simulink model "snap_adc5g_spec"  (R2019a)
settings: Solver=VariableStepDiscrete  StartTime=0.0  StopTime=10.0  RelTol=1e-3
undefined symbols (not defined in the file): pfb_coeff_gen_calc
libraries: xbsIndex_r4 x13965, casper_library_misc x80, casper_library_delays x43, xps_library x5, xbsReplacements_r4 x2, casper_library_communications x1
(part 53 of 152)

== system snap_adc5g_spec/fft_wideband_real/fft_direct/butterfly0_0/bus_convert/conv4 ==
  din : Inport
  all_0s : xbsIndex_r4/Logical  logical_function=NAND  inputs=3  en=off  latency=1  precision=Full  arith_type=Unsigned  n_bits=16  bin_pt=0  align_bp=on  dbl_ovrd=off  block_type=logical
  all_1s : xbsIndex_r4/Logical  logical_function=NAND  inputs=3  en=off  latency=1  precision=Full  arith_type=Unsigned  n_bits=16  bin_pt=0  align_bp=on  dbl_ovrd=off  block_type=logical
  and : xbsIndex_r4/Logical  logical_function=AND  inputs=2  en=off  latency=0  precision=Full  arith_type=Unsigned  n_bits=16  bin_pt=0  align_bp=on  dbl_ovrd=off  block_type=logical
  convert : Subsystem  AncestorBlock=casper_library_misc/convert  mask(convert){bin_pt_in=binary_point_i, n_bits_out=bit_width_o, bin_pt_out=binary_point_o, quantization=Round  (unbiased: Even Values), overflow=Wrap, csp_latency=csp_latency}
      mask prompts: bin_pt_in "Binary Point In"; n_bits_out "Bit Width Out"; bin_pt_out "Binary Point Out"; csp_latency "Latency"
      mask help:
      | Convert input value to the specified bit width and precision.
      |
      | Does not support upscaling number of fractional bits (eg 8_5 to 8_4 is ok, but not 8_4 to 8_5).
      mask init: same as snap_adc5g_spec/fft_wideband_real/fft_direct/butterfly0_0/bus_norm1/conv1
      settings: AttributesFormatString=|
      | N_18 ==> 18_17
      | round even, wrap
      | latency = 1
      mask Help:
      | <pre>
      | Description::
      | 
      | Outputs converted version of the input.
      | 
      | Mask Parameters::
      | 
      | Binary Point In (bin_pt_in): Specifies the binary point location in the input.
      | 
      | Bit Width Out (n_bits_out): Specifies the width of the output.
      | 
      | Binary Point Out (bin_pt_out): Specifies the binary point location in the output.
      | 
      | Quantization (quantization): Specifies quantization handling.
      | 
      | Overflow (overflow): Specifies overflow handling.
      | 
      | Latency (latency): Specifies the latency of the underlying adder block, which is the overall
      | latency of this block as well.
      | </pre>
      mask TypeOptions quantization: Truncate | Round  (unbiased: +/- Inf) | Round  (unbiased: Even Values) | Round  (unbiased: Zero) | Round  (unbiased: Odd Values) | Round  (biased: Up) | Round  (biased: Down)
      mask TypeOptions overflow: Wrap | Saturate | Error
  invert1 : xbsIndex_r4/Inverter  en=off  latency=0  dbl_ovrd=off  block_type=inv
  invert2 : xbsIndex_r4/Inverter  en=off  latency=0  dbl_ovrd=off  block_type=inv
  invert3 : xbsIndex_r4/Inverter  en=off  latency=0  dbl_ovrd=off  block_type=inv
  slice1 : xbsIndex_r4/Slice  nbits=1  boolean_output=on  mode=Upper Bit Location + Width  bit1=0  base1=MSB of Input  bit0=0  base0=LSB of Input  dbl_ovrd=off  block_type=slice
  slice2 : xbsIndex_r4/Slice  nbits=1  boolean_output=on  mode=Upper Bit Location + Width  bit1=-1  base1=MSB of Input  bit0=0  base0=LSB of Input  dbl_ovrd=off  block_type=slice
  slice3 : xbsIndex_r4/Slice  nbits=1  boolean_output=on  mode=Upper Bit Location + Width  bit1=-2  base1=MSB of Input  bit0=0  base0=LSB of Input  dbl_ovrd=off  block_type=slice
  dout : Outport
  of : Outport  Port=2
  wires:
  din/1 -> convert/1(in), slice1/1, slice2/1, slice3/1
  convert/1(out) -> dout/1
  slice1/1 -> all_1s/1, invert1/1
  invert1/1 -> all_0s/1
  slice2/1 -> all_1s/2, invert2/1
  invert2/1 -> all_0s/2
  slice3/1 -> all_1s/3, invert3/1
  invert3/1 -> all_0s/3
  all_0s/1 -> and/1
  all_1s/1 -> and/2
  and/1 -> of/1

== system snap_adc5g_spec/fft_wideband_real/fft_direct/butterfly0_0/bus_convert/conv5 ==
  din : Inport
  all_0s : xbsIndex_r4/Logical  logical_function=NAND  inputs=3  en=off  latency=1  precision=Full  arith_type=Unsigned  n_bits=16  bin_pt=0  align_bp=on  dbl_ovrd=off  block_type=logical
  all_1s : xbsIndex_r4/Logical  logical_function=NAND  inputs=3  en=off  latency=1  precision=Full  arith_type=Unsigned  n_bits=16  bin_pt=0  align_bp=on  dbl_ovrd=off  block_type=logical
  and : xbsIndex_r4/Logical  logical_function=AND  inputs=2  en=off  latency=0  precision=Full  arith_type=Unsigned  n_bits=16  bin_pt=0  align_bp=on  dbl_ovrd=off  block_type=logical
  convert : Subsystem  AncestorBlock=casper_library_misc/convert  mask(convert){bin_pt_in=binary_point_i, n_bits_out=bit_width_o, bin_pt_out=binary_point_o, quantization=Round  (unbiased: Even Values), overflow=Wrap, csp_latency=csp_latency}
      mask prompts: bin_pt_in "Binary Point In"; n_bits_out "Bit Width Out"; bin_pt_out "Binary Point Out"; csp_latency "Latency"
      mask help:
      | Convert input value to the specified bit width and precision.
      |
      | Does not support upscaling number of fractional bits (eg 8_5 to 8_4 is ok, but not 8_4 to 8_5).
      mask init: same as snap_adc5g_spec/fft_wideband_real/fft_direct/butterfly0_0/bus_norm1/conv1
      settings: AttributesFormatString=|
      | N_18 ==> 18_17
      | round even, wrap
      | latency = 1
      mask Help:
      | <pre>
      | Description::
      | 
      | Outputs converted version of the input.
      | 
      | Mask Parameters::
      | 
      | Binary Point In (bin_pt_in): Specifies the binary point location in the input.
      | 
      | Bit Width Out (n_bits_out): Specifies the width of the output.
      | 
      | Binary Point Out (bin_pt_out): Specifies the binary point location in the output.
      | 
      | Quantization (quantization): Specifies quantization handling.
      | 
      | Overflow (overflow): Specifies overflow handling.
      | 
      | Latency (latency): Specifies the latency of the underlying adder block, which is the overall
      | latency of this block as well.
      | </pre>
      mask TypeOptions quantization: Truncate | Round  (unbiased: +/- Inf) | Round  (unbiased: Even Values) | Round  (unbiased: Zero) | Round  (unbiased: Odd Values) | Round  (biased: Up) | Round  (biased: Down)
      mask TypeOptions overflow: Wrap | Saturate | Error
  invert1 : xbsIndex_r4/Inverter  en=off  latency=0  dbl_ovrd=off  block_type=inv
  invert2 : xbsIndex_r4/Inverter  en=off  latency=0  dbl_ovrd=off  block_type=inv
  invert3 : xbsIndex_r4/Inverter  en=off  latency=0  dbl_ovrd=off  block_type=inv
  slice1 : xbsIndex_r4/Slice  nbits=1  boolean_output=on  mode=Upper Bit Location + Width  bit1=0  base1=MSB of Input  bit0=0  base0=LSB of Input  dbl_ovrd=off  block_type=slice
  slice2 : xbsIndex_r4/Slice  nbits=1  boolean_output=on  mode=Upper Bit Location + Width  bit1=-1  base1=MSB of Input  bit0=0  base0=LSB of Input  dbl_ovrd=off  block_type=slice
  slice3 : xbsIndex_r4/Slice  nbits=1  boolean_output=on  mode=Upper Bit Location + Width  bit1=-2  base1=MSB of Input  bit0=0  base0=LSB of Input  dbl_ovrd=off  block_type=slice
  dout : Outport
  of : Outport  Port=2
  wires:
  din/1 -> convert/1(in), slice1/1, slice2/1, slice3/1
  convert/1(out) -> dout/1
  slice1/1 -> all_1s/1, invert1/1
  invert1/1 -> all_0s/1
  slice2/1 -> all_1s/2, invert2/1
  invert2/1 -> all_0s/2
  slice3/1 -> all_1s/3, invert3/1
  invert3/1 -> all_0s/3
  all_0s/1 -> and/1
  all_1s/1 -> and/2
  and/1 -> of/1

== system snap_adc5g_spec/fft_wideband_real/fft_direct/butterfly0_0/bus_convert/conv6 ==
  din : Inport
  all_0s : xbsIndex_r4/Logical  logical_function=NAND  inputs=3  en=off  latency=1  precision=Full  arith_type=Unsigned  n_bits=16  bin_pt=0  align_bp=on  dbl_ovrd=off  block_type=logical
  all_1s : xbsIndex_r4/Logical  logical_function=NAND  inputs=3  en=off  latency=1  precision=Full  arith_type=Unsigned  n_bits=16  bin_pt=0  align_bp=on  dbl_ovrd=off  block_type=logical
  and : xbsIndex_r4/Logical  logical_function=AND  inputs=2  en=off  latency=0  precision=Full  arith_type=Unsigned  n_bits=16  bin_pt=0  align_bp=on  dbl_ovrd=off  block_type=logical
  convert : Subsystem  AncestorBlock=casper_library_misc/convert  mask(convert){bin_pt_in=binary_point_i, n_bits_out=bit_width_o, bin_pt_out=binary_point_o, quantization=Round  (unbiased: Even Values), overflow=Wrap, csp_latency=csp_latency}
      mask prompts: bin_pt_in "Binary Point In"; n_bits_out "Bit Width Out"; bin_pt_out "Binary Point Out"; csp_latency "Latency"
      mask help:
      | Convert input value to the specified bit width and precision.
      |
      | Does not support upscaling number of fractional bits (eg 8_5 to 8_4 is ok, but not 8_4 to 8_5).
      mask init: same as snap_adc5g_spec/fft_wideband_real/fft_direct/butterfly0_0/bus_norm1/conv1
      settings: AttributesFormatString=|
      | N_18 ==> 18_17
      | round even, wrap
      | latency = 1
      mask Help:
      | <pre>
      | Description::
      | 
      | Outputs converted version of the input.
      | 
      | Mask Parameters::
      | 
      | Binary Point In (bin_pt_in): Specifies the binary point location in the input.
      | 
      | Bit Width Out (n_bits_out): Specifies the width of the output.
      | 
      | Binary Point Out (bin_pt_out): Specifies the binary point location in the output.
      | 
      | Quantization (quantization): Specifies quantization handling.
      | 
      | Overflow (overflow): Specifies overflow handling.
      | 
      | Latency (latency): Specifies the latency of the underlying adder block, which is the overall
      | latency of this block as well.
      | </pre>
      mask TypeOptions quantization: Truncate | Round  (unbiased: +/- Inf) | Round  (unbiased: Even Values) | Round  (unbiased: Zero) | Round  (unbiased: Odd Values) | Round  (biased: Up) | Round  (biased: Down)
      mask TypeOptions overflow: Wrap | Saturate | Error
  invert1 : xbsIndex_r4/Inverter  en=off  latency=0  dbl_ovrd=off  block_type=inv
  invert2 : xbsIndex_r4/Inverter  en=off  latency=0  dbl_ovrd=off  block_type=inv
  invert3 : xbsIndex_r4/Inverter  en=off  latency=0  dbl_ovrd=off  block_type=inv
  slice1 : xbsIndex_r4/Slice  nbits=1  boolean_output=on  mode=Upper Bit Location + Width  bit1=0  base1=MSB of Input  bit0=0  base0=LSB of Input  dbl_ovrd=off  block_type=slice
  slice2 : xbsIndex_r4/Slice  nbits=1  boolean_output=on  mode=Upper Bit Location + Width  bit1=-1  base1=MSB of Input  bit0=0  base0=LSB of Input  dbl_ovrd=off  block_type=slice
  slice3 : xbsIndex_r4/Slice  nbits=1  boolean_output=on  mode=Upper Bit Location + Width  bit1=-2  base1=MSB of Input  bit0=0  base0=LSB of Input  dbl_ovrd=off  block_type=slice
  dout : Outport
  of : Outport  Port=2
  wires:
  din/1 -> convert/1(in), slice1/1, slice2/1, slice3/1
  convert/1(out) -> dout/1
  slice1/1 -> all_1s/1, invert1/1
  invert1/1 -> all_0s/1
  slice2/1 -> all_1s/2, invert2/1
  invert2/1 -> all_0s/2
  slice3/1 -> all_1s/3, invert3/1
  invert3/1 -> all_0s/3
  all_0s/1 -> and/1
  all_1s/1 -> and/2
  and/1 -> of/1

== system snap_adc5g_spec/fft_wideband_real/fft_direct/butterfly0_0/bus_convert/conv7 ==
  din : Inport
  all_0s : xbsIndex_r4/Logical  logical_function=NAND  inputs=3  en=off  latency=1  precision=Full  arith_type=Unsigned  n_bits=16  bin_pt=0  align_bp=on  dbl_ovrd=off  block_type=logical
  all_1s : xbsIndex_r4/Logical  logical_function=NAND  inputs=3  en=off  latency=1  precision=Full  arith_type=Unsigned  n_bits=16  bin_pt=0  align_bp=on  dbl_ovrd=off  block_type=logical
  and : xbsIndex_r4/Logical  logical_function=AND  inputs=2  en=off  latency=0  precision=Full  arith_type=Unsigned  n_bits=16  bin_pt=0  align_bp=on  dbl_ovrd=off  block_type=logical
  convert : Subsystem  AncestorBlock=casper_library_misc/convert  mask(convert){bin_pt_in=binary_point_i, n_bits_out=bit_width_o, bin_pt_out=binary_point_o, quantization=Round  (unbiased: Even Values), overflow=Wrap, csp_latency=csp_latency}
      mask prompts: bin_pt_in "Binary Point In"; n_bits_out "Bit Width Out"; bin_pt_out "Binary Point Out"; csp_latency "Latency"
      mask help:
      | Convert input value to the specified bit width and precision.
      |
      | Does not support upscaling number of fractional bits (eg 8_5 to 8_4 is ok, but not 8_4 to 8_5).
      mask init: same as snap_adc5g_spec/fft_wideband_real/fft_direct/butterfly0_0/bus_norm1/conv1
      settings: AttributesFormatString=|
      | N_18 ==> 18_17
      | round even, wrap
      | latency = 1
      mask Help:
      | <pre>
      | Description::
      | 
      | Outputs converted version of the input.
      | 
      | Mask Parameters::
      | 
      | Binary Point In (bin_pt_in): Specifies the binary point location in the input.
      | 
      | Bit Width Out (n_bits_out): Specifies the width of the output.
      | 
      | Binary Point Out (bin_pt_out): Specifies the binary point location in the output.
      | 
      | Quantization (quantization): Specifies quantization handling.
      | 
      | Overflow (overflow): Specifies overflow handling.
      | 
      | Latency (latency): Specifies the latency of the underlying adder block, which is the overall
      | latency of this block as well.
      | </pre>
      mask TypeOptions quantization: Truncate | Round  (unbiased: +/- Inf) | Round  (unbiased: Even Values) | Round  (unbiased: Zero) | Round  (unbiased: Odd Values) | Round  (biased: Up) | Round  (biased: Down)
      mask TypeOptions overflow: Wrap | Saturate | Error
  invert1 : xbsIndex_r4/Inverter  en=off  latency=0  dbl_ovrd=off  block_type=inv
  invert2 : xbsIndex_r4/Inverter  en=off  latency=0  dbl_ovrd=off  block_type=inv
  invert3 : xbsIndex_r4/Inverter  en=off  latency=0  dbl_ovrd=off  block_type=inv
  slice1 : xbsIndex_r4/Slice  nbits=1  boolean_output=on  mode=Upper Bit Location + Width  bit1=0  base1=MSB of Input  bit0=0  base0=LSB of Input  dbl_ovrd=off  block_type=slice
  slice2 : xbsIndex_r4/Slice  nbits=1  boolean_output=on  mode=Upper Bit Location + Width  bit1=-1  base1=MSB of Input  bit0=0  base0=LSB of Input  dbl_ovrd=off  block_type=slice
  slice3 : xbsIndex_r4/Slice  nbits=1  boolean_output=on  mode=Upper Bit Location + Width  bit1=-2  base1=MSB of Input  bit0=0  base0=LSB of Input  dbl_ovrd=off  block_type=slice
  dout : Outport
  of : Outport  Port=2
  wires:
  din/1 -> convert/1(in), slice1/1, slice2/1, slice3/1
  convert/1(out) -> dout/1
  slice1/1 -> all_1s/1, invert1/1
  invert1/1 -> all_0s/1
  slice2/1 -> all_1s/2, invert2/1
  invert2/1 -> all_0s/2
  slice3/1 -> all_1s/3, invert3/1
  invert3/1 -> all_0s/3
  all_0s/1 -> and/1
  all_1s/1 -> and/2
  and/1 -> of/1

== system snap_adc5g_spec/fft_wideband_real/fft_direct/butterfly0_0/bus_convert/conv8 ==
  din : Inport
  all_0s : xbsIndex_r4/Logical  logical_function=NAND  inputs=3  en=off  latency=1  precision=Full  arith_type=Unsigned  n_bits=16  bin_pt=0  align_bp=on  dbl_ovrd=off  block_type=logical
  all_1s : xbsIndex_r4/Logical  logical_function=NAND  inputs=3  en=off  latency=1  precision=Full  arith_type=Unsigned  n_bits=16  bin_pt=0  align_bp=on  dbl_ovrd=off  block_type=logical
  and : xbsIndex_r4/Logical  logical_function=AND  inputs=2  en=off  latency=0  precision=Full  arith_type=Unsigned  n_bits=16  bin_pt=0  align_bp=on  dbl_ovrd=off  block_type=logical
  convert : Subsystem  AncestorBlock=casper_library_misc/convert  mask(convert){bin_pt_in=binary_point_i, n_bits_out=bit_width_o, bin_pt_out=binary_point_o, quantization=Round  (unbiased: Even Values), overflow=Wrap, csp_latency=csp_latency}
      mask prompts: bin_pt_in "Binary Point In"; n_bits_out "Bit Width Out"; bin_pt_out "Binary Point Out"; csp_latency "Latency"
      mask help:
      | Convert input value to the specified bit width and precision.
      |
      | Does not support upscaling number of fractional bits (eg 8_5 to 8_4 is ok, but not 8_4 to 8_5).
      mask init: same as snap_adc5g_spec/fft_wideband_real/fft_direct/butterfly0_0/bus_norm1/conv1
      settings: AttributesFormatString=|
      | N_18 ==> 18_17
      | round even, wrap
      | latency = 1
      mask Help:
      | <pre>
      | Description::
      | 
      | Outputs converted version of the input.
      | 
      | Mask Parameters::
      | 
      | Binary Point In (bin_pt_in): Specifies the binary point location in the input.
      | 
      | Bit Width Out (n_bits_out): Specifies the width of the output.
      | 
      | Binary Point Out (bin_pt_out): Specifies the binary point location in the output.
      | 
      | Quantization (quantization): Specifies quantization handling.
      | 
      | Overflow (overflow): Specifies overflow handling.
      | 
      | Latency (latency): Specifies the latency of the underlying adder block, which is the overall
      | latency of this block as well.
      | </pre>
      mask TypeOptions quantization: Truncate | Round  (unbiased: +/- Inf) | Round  (unbiased: Even Values) | Round  (unbiased: Zero) | Round  (unbiased: Odd Values) | Round  (biased: Up) | Round  (biased: Down)
      mask TypeOptions overflow: Wrap | Saturate | Error
  invert1 : xbsIndex_r4/Inverter  en=off  latency=0  dbl_ovrd=off  block_type=inv
  invert2 : xbsIndex_r4/Inverter  en=off  latency=0  dbl_ovrd=off  block_type=inv
  invert3 : xbsIndex_r4/Inverter  en=off  latency=0  dbl_ovrd=off  block_type=inv
  slice1 : xbsIndex_r4/Slice  nbits=1  boolean_output=on  mode=Upper Bit Location + Width  bit1=0  base1=MSB of Input  bit0=0  base0=LSB of Input  dbl_ovrd=off  block_type=slice
  slice2 : xbsIndex_r4/Slice  nbits=1  boolean_output=on  mode=Upper Bit Location + Width  bit1=-1  base1=MSB of Input  bit0=0  base0=LSB of Input  dbl_ovrd=off  block_type=slice
  slice3 : xbsIndex_r4/Slice  nbits=1  boolean_output=on  mode=Upper Bit Location + Width  bit1=-2  base1=MSB of Input  bit0=0  base0=LSB of Input  dbl_ovrd=off  block_type=slice
  dout : Outport
  of : Outport  Port=2
  wires:
  din/1 -> convert/1(in), slice1/1, slice2/1, slice3/1
  convert/1(out) -> dout/1
  slice1/1 -> all_1s/1, invert1/1
  invert1/1 -> all_0s/1
  slice2/1 -> all_1s/2, invert2/1
  invert2/1 -> all_0s/2
  slice3/1 -> all_1s/3, invert3/1
  invert3/1 -> all_0s/3
  all_0s/1 -> and/1
  all_1s/1 -> and/2
  and/1 -> of/1

== system snap_adc5g_spec/fft_wideband_real/fft_direct/butterfly0_0/bus_convert/conv9 ==
  din : Inport
  all_0s : xbsIndex_r4/Logical  logical_function=NAND  inputs=3  en=off  latency=1  precision=Full  arith_type=Unsigned  n_bits=16  bin_pt=0  align_bp=on  dbl_ovrd=off  block_type=logical
  all_1s : xbsIndex_r4/Logical  logical_function=NAND  inputs=3  en=off  latency=1  precision=Full  arith_type=Unsigned  n_bits=16  bin_pt=0  align_bp=on  dbl_ovrd=off  block_type=logical
  and : xbsIndex_r4/Logical  logical_function=AND  inputs=2  en=off  latency=0  precision=Full  arith_type=Unsigned  n_bits=16  bin_pt=0  align_bp=on  dbl_ovrd=off  block_type=logical
  convert : Subsystem  AncestorBlock=casper_library_misc/convert  mask(convert){bin_pt_in=binary_point_i, n_bits_out=bit_width_o, bin_pt_out=binary_point_o, quantization=Round  (unbiased: Even Values), overflow=Wrap, csp_latency=csp_latency}
      mask prompts: bin_pt_in "Binary Point In"; n_bits_out "Bit Width Out"; bin_pt_out "Binary Point Out"; csp_latency "Latency"
      mask help:
      | Convert input value to the specified bit width and precision.
      |
      | Does not support upscaling number of fractional bits (eg 8_5 to 8_4 is ok, but not 8_4 to 8_5).
      mask init: same as snap_adc5g_spec/fft_wideband_real/fft_direct/butterfly0_0/bus_norm1/conv1
      settings: AttributesFormatString=|
      | N_18 ==> 18_17
      | round even, wrap
      | latency = 1
      mask Help:
      | <pre>
      | Description::
      | 
      | Outputs converted version of the input.
      | 
      | Mask Parameters::
      | 
      | Binary Point In (bin_pt_in): Specifies the binary point location in the input.
      | 
      | Bit Width Out (n_bits_out): Specifies the width of the output.
      | 
      | Binary Point Out (bin_pt_out): Specifies the binary point location in the output.
      | 
      | Quantization (quantization): Specifies quantization handling.
      | 
      | Overflow (overflow): Specifies overflow handling.
      | 
      | Latency (latency): Specifies the latency of the underlying adder block, which is the overall
      | latency of this block as well.
      | </pre>
      mask TypeOptions quantization: Truncate | Round  (unbiased: +/- Inf) | Round  (unbiased: Even Values) | Round  (unbiased: Zero) | Round  (unbiased: Odd Values) | Round  (biased: Up) | Round  (biased: Down)
      mask TypeOptions overflow: Wrap | Saturate | Error
  invert1 : xbsIndex_r4/Inverter  en=off  latency=0  dbl_ovrd=off  block_type=inv
  invert2 : xbsIndex_r4/Inverter  en=off  latency=0  dbl_ovrd=off  block_type=inv
  invert3 : xbsIndex_r4/Inverter  en=off  latency=0  dbl_ovrd=off  block_type=inv
  slice1 : xbsIndex_r4/Slice  nbits=1  boolean_output=on  mode=Upper Bit Location + Width  bit1=0  base1=MSB of Input  bit0=0  base0=LSB of Input  dbl_ovrd=off  block_type=slice
  slice2 : xbsIndex_r4/Slice  nbits=1  boolean_output=on  mode=Upper Bit Location + Width  bit1=-1  base1=MSB of Input  bit0=0  base0=LSB of Input  dbl_ovrd=off  block_type=slice
  slice3 : xbsIndex_r4/Slice  nbits=1  boolean_output=on  mode=Upper Bit Location + Width  bit1=-2  base1=MSB of Input  bit0=0  base0=LSB of Input  dbl_ovrd=off  block_type=slice
  dout : Outport
  of : Outport  Port=2
  wires:
  din/1 -> convert/1(in), slice1/1, slice2/1, slice3/1
  convert/1(out) -> dout/1
  slice1/1 -> all_1s/1, invert1/1
  invert1/1 -> all_0s/1
  slice2/1 -> all_1s/2, invert2/1
  invert2/1 -> all_0s/2
  slice3/1 -> all_1s/3, invert3/1
  invert3/1 -> all_0s/3
  all_0s/1 -> and/1
  all_1s/1 -> and/2
  and/1 -> of/1

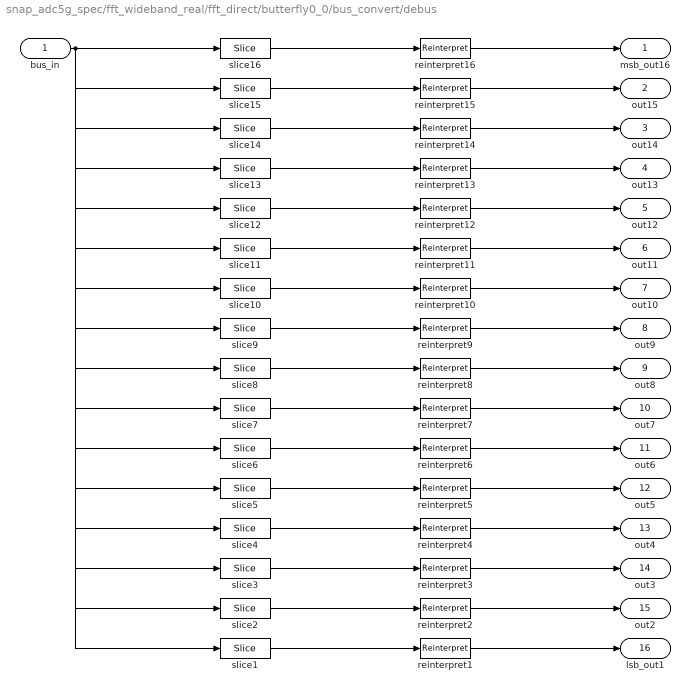
== system snap_adc5g_spec/fft_wideband_real/fft_direct/butterfly0_0/bus_convert/debus ==
  bus_in : Inport
  reinterpret{1..16} (16 alike) : xbsIndex_r4/Reinterpret  force_arith_type=on  arith_type="Signed  (2's comp)"  force_bin_pt=on  bin_pt=18  block_type=reinterpret
  slice1 : xbsIndex_r4/Slice  nbits=21  boolean_output=off  mode=Upper Bit Location + Width  bit1=-315  base1=MSB of Input  bit0=0  base0=LSB of Input  dbl_ovrd=off  block_type=slice
  slice10 : xbsIndex_r4/Slice  nbits=21  boolean_output=off  mode=Upper Bit Location + Width  bit1=-126  base1=MSB of Input  bit0=0  base0=LSB of Input  dbl_ovrd=off  block_type=slice
  slice11 : xbsIndex_r4/Slice  nbits=21  boolean_output=off  mode=Upper Bit Location + Width  bit1=-105  base1=MSB of Input  bit0=0  base0=LSB of Input  dbl_ovrd=off  block_type=slice
  slice12 : xbsIndex_r4/Slice  nbits=21  boolean_output=off  mode=Upper Bit Location + Width  bit1=-84  base1=MSB of Input  bit0=0  base0=LSB of Input  dbl_ovrd=off  block_type=slice
  slice13 : xbsIndex_r4/Slice  nbits=21  boolean_output=off  mode=Upper Bit Location + Width  bit1=-63  base1=MSB of Input  bit0=0  base0=LSB of Input  dbl_ovrd=off  block_type=slice
  slice14 : xbsIndex_r4/Slice  nbits=21  boolean_output=off  mode=Upper Bit Location + Width  bit1=-42  base1=MSB of Input  bit0=0  base0=LSB of Input  dbl_ovrd=off  block_type=slice
  slice15 : xbsIndex_r4/Slice  nbits=21  boolean_output=off  mode=Upper Bit Location + Width  bit1=-21  base1=MSB of Input  bit0=0  base0=LSB of Input  dbl_ovrd=off  block_type=slice
  slice16 : xbsIndex_r4/Slice  nbits=21  boolean_output=off  mode=Upper Bit Location + Width  bit1=0  base1=MSB of Input  bit0=0  base0=LSB of Input  dbl_ovrd=off  block_type=slice
  slice2 : xbsIndex_r4/Slice  nbits=21  boolean_output=off  mode=Upper Bit Location + Width  bit1=-294  base1=MSB of Input  bit0=0  base0=LSB of Input  dbl_ovrd=off  block_type=slice
  slice3 : xbsIndex_r4/Slice  nbits=21  boolean_output=off  mode=Upper Bit Location + Width  bit1=-273  base1=MSB of Input  bit0=0  base0=LSB of Input  dbl_ovrd=off  block_type=slice
  slice4 : xbsIndex_r4/Slice  nbits=21  boolean_output=off  mode=Upper Bit Location + Width  bit1=-252  base1=MSB of Input  bit0=0  base0=LSB of Input  dbl_ovrd=off  block_type=slice
  slice5 : xbsIndex_r4/Slice  nbits=21  boolean_output=off  mode=Upper Bit Location + Width  bit1=-231  base1=MSB of Input  bit0=0  base0=LSB of Input  dbl_ovrd=off  block_type=slice
  slice6 : xbsIndex_r4/Slice  nbits=21  boolean_output=off  mode=Upper Bit Location + Width  bit1=-210  base1=MSB of Input  bit0=0  base0=LSB of Input  dbl_ovrd=off  block_type=slice
  slice7 : xbsIndex_r4/Slice  nbits=21  boolean_output=off  mode=Upper Bit Location + Width  bit1=-189  base1=MSB of Input  bit0=0  base0=LSB of Input  dbl_ovrd=off  block_type=slice
  slice8 : xbsIndex_r4/Slice  nbits=21  boolean_output=off  mode=Upper Bit Location + Width  bit1=-168  base1=MSB of Input  bit0=0  base0=LSB of Input  dbl_ovrd=off  block_type=slice
  slice9 : xbsIndex_r4/Slice  nbits=21  boolean_output=off  mode=Upper Bit Location + Width  bit1=-147  base1=MSB of Input  bit0=0  base0=LSB of Input  dbl_ovrd=off  block_type=slice
  msb_out16 : Outport
  out15 : Outport  Port=2
  out14 : Outport  Port=3
  out13 : Outport  Port=4
  out12 : Outport  Port=5
  out11 : Outport  Port=6
  out10 : Outport  Port=7
  out9 : Outport  Port=8
  out8 : Outport  Port=9
  out7 : Outport  Port=10
  out6 : Outport  Port=11
  out5 : Outport  Port=12
  out4 : Outport  Port=13
  out3 : Outport  Port=14
  out2 : Outport  Port=15
  lsb_out1 : Outport  Port=16
  wires:
  bus_in/1 -> slice16/1, slice15/1, slice14/1, slice13/1, slice12/1, slice11/1, slice10/1, slice9/1, slice8/1, slice7/1, slice6/1, slice5/1, slice4/1, slice3/1, slice2/1, slice1/1
  slice16/1 -> reinterpret16/1
  reinterpret16/1 -> msb_out16/1
  slice15/1 -> reinterpret15/1
  reinterpret15/1 -> out15/1
  slice14/1 -> reinterpret14/1
  reinterpret14/1 -> out14/1
  slice13/1 -> reinterpret13/1
  reinterpret13/1 -> out13/1
  slice12/1 -> reinterpret12/1
  reinterpret12/1 -> out12/1
  slice11/1 -> reinterpret11/1
  reinterpret11/1 -> out11/1
  slice10/1 -> reinterpret10/1
  reinterpret10/1 -> out10/1
  slice9/1 -> reinterpret9/1
  reinterpret9/1 -> out9/1
  slice8/1 -> reinterpret8/1
  reinterpret8/1 -> out8/1
  slice7/1 -> reinterpret7/1
  reinterpret7/1 -> out7/1
  slice6/1 -> reinterpret6/1
  reinterpret6/1 -> out6/1
  slice5/1 -> reinterpret5/1
  reinterpret5/1 -> out5/1
  slice4/1 -> reinterpret4/1
  reinterpret4/1 -> out4/1
  slice3/1 -> reinterpret3/1
  reinterpret3/1 -> out3/1
  slice2/1 -> reinterpret2/1
  reinterpret2/1 -> out2/1
  slice1/1 -> reinterpret1/1
  reinterpret1/1 -> lsb_out1/1

== system snap_adc5g_spec/fft_wideband_real/fft_direct/butterfly0_0/bus_convert/of_bussify ==
  in1 : Inport
  in2 : Inport  Port=2
  in3 : Inport  Port=3
  in4 : Inport  Port=4
  in5 : Inport  Port=5
  in6 : Inport  Port=6
  in7 : Inport  Port=7
  in8 : Inport  Port=8
  in9 : Inport  Port=9
  in10 : Inport  Port=10
  in11 : Inport  Port=11
  in12 : Inport  Port=12
  in13 : Inport  Port=13
  in14 : Inport  Port=14
  in15 : Inport  Port=15
  in16 : Inport  Port=16
  concatenate : xbsIndex_r4/Concat  num_inputs=16  dbl_ovrd=off  block_type=concat
  reinterpret{1..16} (16 alike) : xbsIndex_r4/Reinterpret  force_arith_type=on  arith_type=Unsigned  force_bin_pt=on  bin_pt=0  block_type=reinterpret
      reinterpret1 settings: infoedit="Changes signal type without altering the binary representation.   You can changed the signal between signed and unsigned, and relocate the binary point.<br><br>Hardware notes: In hardware this block costs nothing.<br><br>Example:  Suppose the input is 6 bits wide, signed, with 2 fractional bits, and the output is forced to unsigned with 0 fractional bits.  Then an input of -2.0 (1110.00 in binary 2's complement) becomes an output of 56 (111000 in binary)."
      reinterpret2 settings: infoedit="Changes signal type without altering the binary representation.   You can changed the signal between signed and unsigned, and relocate the binary point.<br><br>Hardware notes: In hardware this block costs nothing.<br><br>Example:  Suppose the input is 6 bits wide, signed, with 2 fractional bits, and the output is forced to unsigned with 0 fractional bits.  Then an input of -2.0 (1110.00 in binary 2's complement) becomes an output of 56 (111000 in binary)."
  bus_out : Outport
  wires:
  concatenate/1 -> bus_out/1
  in1/1 -> reinterpret1/1
  reinterpret1/1 -> concatenate/1
  in2/1 -> reinterpret2/1
  reinterpret2/1 -> concatenate/2
  in3/1 -> reinterpret3/1
  reinterpret3/1 -> concatenate/3
  in4/1 -> reinterpret4/1
  reinterpret4/1 -> concatenate/4
  in5/1 -> reinterpret5/1
  reinterpret5/1 -> concatenate/5
  in6/1 -> reinterpret6/1
  reinterpret6/1 -> concatenate/6
  in7/1 -> reinterpret7/1
  reinterpret7/1 -> concatenate/7
  in8/1 -> reinterpret8/1
  reinterpret8/1 -> concatenate/8
  in9/1 -> reinterpret9/1
  reinterpret9/1 -> concatenate/9
  in10/1 -> reinterpret10/1
  reinterpret10/1 -> concatenate/10
  in11/1 -> reinterpret11/1
  reinterpret11/1 -> concatenate/11
  in12/1 -> reinterpret12/1
  reinterpret12/1 -> concatenate/12
  in13/1 -> reinterpret13/1
  reinterpret13/1 -> concatenate/13
  in14/1 -> reinterpret14/1
  reinterpret14/1 -> concatenate/14
  in15/1 -> reinterpret15/1
  reinterpret15/1 -> concatenate/15
  in16/1 -> reinterpret16/1
  reinterpret16/1 -> concatenate/16

== system snap_adc5g_spec/fft_wideband_real/fft_direct/butterfly0_0/bus_norm0/bussify ==
  in1 : Inport
  in2 : Inport  Port=2
  in3 : Inport  Port=3
  in4 : Inport  Port=4
  in5 : Inport  Port=5
  in6 : Inport  Port=6
  in7 : Inport  Port=7
  in8 : Inport  Port=8
  in9 : Inport  Port=9
  in10 : Inport  Port=10
  in11 : Inport  Port=11
  in12 : Inport  Port=12
  in13 : Inport  Port=13
  in14 : Inport  Port=14
  in15 : Inport  Port=15
  in16 : Inport  Port=16
  concatenate : xbsIndex_r4/Concat  num_inputs=16  dbl_ovrd=off  block_type=concat
  reinterpret{1..16} (16 alike) : xbsIndex_r4/Reinterpret  force_arith_type=on  arith_type=Unsigned  force_bin_pt=on  bin_pt=0  block_type=reinterpret
      reinterpret1 settings: infoedit="Changes signal type without altering the binary representation.   You can changed the signal between signed and unsigned, and relocate the binary point.<br><br>Hardware notes: In hardware this block costs nothing.<br><br>Example:  Suppose the input is 6 bits wide, signed, with 2 fractional bits, and the output is forced to unsigned with 0 fractional bits.  Then an input of -2.0 (1110.00 in binary 2's complement) becomes an output of 56 (111000 in binary)."
      reinterpret2 settings: infoedit="Changes signal type without altering the binary representation.   You can changed the signal between signed and unsigned, and relocate the binary point.<br><br>Hardware notes: In hardware this block costs nothing.<br><br>Example:  Suppose the input is 6 bits wide, signed, with 2 fractional bits, and the output is forced to unsigned with 0 fractional bits.  Then an input of -2.0 (1110.00 in binary 2's complement) becomes an output of 56 (111000 in binary)."
  bus_out : Outport
  wires:
  concatenate/1 -> bus_out/1
  in1/1 -> reinterpret1/1
  reinterpret1/1 -> concatenate/1
  in2/1 -> reinterpret2/1
  reinterpret2/1 -> concatenate/2
  in3/1 -> reinterpret3/1
  reinterpret3/1 -> concatenate/3
  in4/1 -> reinterpret4/1
  reinterpret4/1 -> concatenate/4
  in5/1 -> reinterpret5/1
  reinterpret5/1 -> concatenate/5
  in6/1 -> reinterpret6/1
  reinterpret6/1 -> concatenate/6
  in7/1 -> reinterpret7/1
  reinterpret7/1 -> concatenate/7
  in8/1 -> reinterpret8/1
  reinterpret8/1 -> concatenate/8
  in9/1 -> reinterpret9/1
  reinterpret9/1 -> concatenate/9
  in10/1 -> reinterpret10/1
  reinterpret10/1 -> concatenate/10
  in11/1 -> reinterpret11/1
  reinterpret11/1 -> concatenate/11
  in12/1 -> reinterpret12/1
  reinterpret12/1 -> concatenate/12
  in13/1 -> reinterpret13/1
  reinterpret13/1 -> concatenate/13
  in14/1 -> reinterpret14/1
  reinterpret14/1 -> concatenate/14
  in15/1 -> reinterpret15/1
  reinterpret15/1 -> concatenate/15
  in16/1 -> reinterpret16/1
  reinterpret16/1 -> concatenate/16

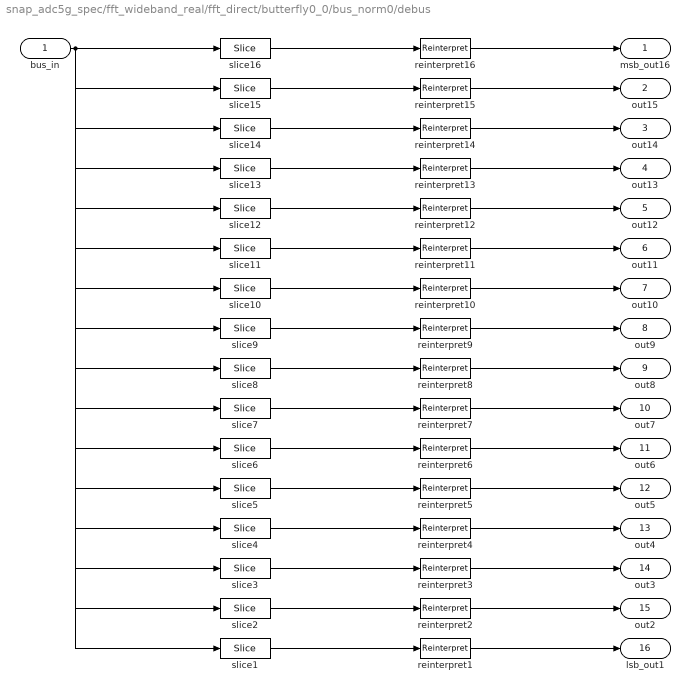
== system snap_adc5g_spec/fft_wideband_real/fft_direct/butterfly0_0/bus_norm0/debus ==
  bus_in : Inport
  reinterpret{1..16} (16 alike) : xbsIndex_r4/Reinterpret  force_arith_type=on  arith_type="Signed  (2's comp)"  force_bin_pt=on  bin_pt=17  block_type=reinterpret
  slice1 : xbsIndex_r4/Slice  nbits=20  boolean_output=off  mode=Upper Bit Location + Width  bit1=-300  base1=MSB of Input  bit0=0  base0=LSB of Input  dbl_ovrd=off  block_type=slice
  slice10 : xbsIndex_r4/Slice  nbits=20  boolean_output=off  mode=Upper Bit Location + Width  bit1=-120  base1=MSB of Input  bit0=0  base0=LSB of Input  dbl_ovrd=off  block_type=slice
  slice11 : xbsIndex_r4/Slice  nbits=20  boolean_output=off  mode=Upper Bit Location + Width  bit1=-100  base1=MSB of Input  bit0=0  base0=LSB of Input  dbl_ovrd=off  block_type=slice
  slice12 : xbsIndex_r4/Slice  nbits=20  boolean_output=off  mode=Upper Bit Location + Width  bit1=-80  base1=MSB of Input  bit0=0  base0=LSB of Input  dbl_ovrd=off  block_type=slice
  slice13 : xbsIndex_r4/Slice  nbits=20  boolean_output=off  mode=Upper Bit Location + Width  bit1=-60  base1=MSB of Input  bit0=0  base0=LSB of Input  dbl_ovrd=off  block_type=slice
  slice14 : xbsIndex_r4/Slice  nbits=20  boolean_output=off  mode=Upper Bit Location + Width  bit1=-40  base1=MSB of Input  bit0=0  base0=LSB of Input  dbl_ovrd=off  block_type=slice
  slice15 : xbsIndex_r4/Slice  nbits=20  boolean_output=off  mode=Upper Bit Location + Width  bit1=-20  base1=MSB of Input  bit0=0  base0=LSB of Input  dbl_ovrd=off  block_type=slice
  slice16 : xbsIndex_r4/Slice  nbits=20  boolean_output=off  mode=Upper Bit Location + Width  bit1=0  base1=MSB of Input  bit0=0  base0=LSB of Input  dbl_ovrd=off  block_type=slice
  slice2 : xbsIndex_r4/Slice  nbits=20  boolean_output=off  mode=Upper Bit Location + Width  bit1=-280  base1=MSB of Input  bit0=0  base0=LSB of Input  dbl_ovrd=off  block_type=slice
  slice3 : xbsIndex_r4/Slice  nbits=20  boolean_output=off  mode=Upper Bit Location + Width  bit1=-260  base1=MSB of Input  bit0=0  base0=LSB of Input  dbl_ovrd=off  block_type=slice
  slice4 : xbsIndex_r4/Slice  nbits=20  boolean_output=off  mode=Upper Bit Location + Width  bit1=-240  base1=MSB of Input  bit0=0  base0=LSB of Input  dbl_ovrd=off  block_type=slice
  slice5 : xbsIndex_r4/Slice  nbits=20  boolean_output=off  mode=Upper Bit Location + Width  bit1=-220  base1=MSB of Input  bit0=0  base0=LSB of Input  dbl_ovrd=off  block_type=slice
  slice6 : xbsIndex_r4/Slice  nbits=20  boolean_output=off  mode=Upper Bit Location + Width  bit1=-200  base1=MSB of Input  bit0=0  base0=LSB of Input  dbl_ovrd=off  block_type=slice
  slice7 : xbsIndex_r4/Slice  nbits=20  boolean_output=off  mode=Upper Bit Location + Width  bit1=-180  base1=MSB of Input  bit0=0  base0=LSB of Input  dbl_ovrd=off  block_type=slice
  slice8 : xbsIndex_r4/Slice  nbits=20  boolean_output=off  mode=Upper Bit Location + Width  bit1=-160  base1=MSB of Input  bit0=0  base0=LSB of Input  dbl_ovrd=off  block_type=slice
  slice9 : xbsIndex_r4/Slice  nbits=20  boolean_output=off  mode=Upper Bit Location + Width  bit1=-140  base1=MSB of Input  bit0=0  base0=LSB of Input  dbl_ovrd=off  block_type=slice
  msb_out16 : Outport
  out15 : Outport  Port=2
  out14 : Outport  Port=3
  out13 : Outport  Port=4
  out12 : Outport  Port=5
  out11 : Outport  Port=6
  out10 : Outport  Port=7
  out9 : Outport  Port=8
  out8 : Outport  Port=9
  out7 : Outport  Port=10
  out6 : Outport  Port=11
  out5 : Outport  Port=12
  out4 : Outport  Port=13
  out3 : Outport  Port=14
  out2 : Outport  Port=15
  lsb_out1 : Outport  Port=16
  wires:
  bus_in/1 -> slice16/1, slice15/1, slice14/1, slice13/1, slice12/1, slice11/1, slice10/1, slice9/1, slice8/1, slice7/1, slice6/1, slice5/1, slice4/1, slice3/1, slice2/1, slice1/1
  slice16/1 -> reinterpret16/1
  reinterpret16/1 -> msb_out16/1
  slice15/1 -> reinterpret15/1
  reinterpret15/1 -> out15/1
  slice14/1 -> reinterpret14/1
  reinterpret14/1 -> out14/1
  slice13/1 -> reinterpret13/1
  reinterpret13/1 -> out13/1
  slice12/1 -> reinterpret12/1
  reinterpret12/1 -> out12/1
  slice11/1 -> reinterpret11/1
  reinterpret11/1 -> out11/1
  slice10/1 -> reinterpret10/1
  reinterpret10/1 -> out10/1
  slice9/1 -> reinterpret9/1
  reinterpret9/1 -> out9/1
  slice8/1 -> reinterpret8/1
  reinterpret8/1 -> out8/1
  slice7/1 -> reinterpret7/1
  reinterpret7/1 -> out7/1
  slice6/1 -> reinterpret6/1
  reinterpret6/1 -> out6/1
  slice5/1 -> reinterpret5/1
  reinterpret5/1 -> out5/1
  slice4/1 -> reinterpret4/1
  reinterpret4/1 -> out4/1
  slice3/1 -> reinterpret3/1
  reinterpret3/1 -> out3/1
  slice2/1 -> reinterpret2/1
  reinterpret2/1 -> out2/1
  slice1/1 -> reinterpret1/1
  reinterpret1/1 -> lsb_out1/1

== system snap_adc5g_spec/fft_wideband_real/fft_direct/butterfly0_0/bus_norm1/bussify ==
  in1 : Inport
  in2 : Inport  Port=2
  in3 : Inport  Port=3
  in4 : Inport  Port=4
  in5 : Inport  Port=5
  in6 : Inport  Port=6
  in7 : Inport  Port=7
  in8 : Inport  Port=8
  in9 : Inport  Port=9
  in10 : Inport  Port=10
  in11 : Inport  Port=11
  in12 : Inport  Port=12
  in13 : Inport  Port=13
  in14 : Inport  Port=14
  in15 : Inport  Port=15
  in16 : Inport  Port=16
  concatenate : xbsIndex_r4/Concat  num_inputs=16  dbl_ovrd=off  block_type=concat
  reinterpret{1..16} (16 alike) : xbsIndex_r4/Reinterpret  force_arith_type=on  arith_type=Unsigned  force_bin_pt=on  bin_pt=0  block_type=reinterpret
      reinterpret1 settings: infoedit="Changes signal type without altering the binary representation.   You can changed the signal between signed and unsigned, and relocate the binary point.<br><br>Hardware notes: In hardware this block costs nothing.<br><br>Example:  Suppose the input is 6 bits wide, signed, with 2 fractional bits, and the output is forced to unsigned with 0 fractional bits.  Then an input of -2.0 (1110.00 in binary 2's complement) becomes an output of 56 (111000 in binary)."
      reinterpret2 settings: infoedit="Changes signal type without altering the binary representation.   You can changed the signal between signed and unsigned, and relocate the binary point.<br><br>Hardware notes: In hardware this block costs nothing.<br><br>Example:  Suppose the input is 6 bits wide, signed, with 2 fractional bits, and the output is forced to unsigned with 0 fractional bits.  Then an input of -2.0 (1110.00 in binary 2's complement) becomes an output of 56 (111000 in binary)."
  bus_out : Outport
  wires:
  concatenate/1 -> bus_out/1
  in1/1 -> reinterpret1/1
  reinterpret1/1 -> concatenate/1
  in2/1 -> reinterpret2/1
  reinterpret2/1 -> concatenate/2
  in3/1 -> reinterpret3/1
  reinterpret3/1 -> concatenate/3
  in4/1 -> reinterpret4/1
  reinterpret4/1 -> concatenate/4
  in5/1 -> reinterpret5/1
  reinterpret5/1 -> concatenate/5
  in6/1 -> reinterpret6/1
  reinterpret6/1 -> concatenate/6
  in7/1 -> reinterpret7/1
  reinterpret7/1 -> concatenate/7
  in8/1 -> reinterpret8/1
  reinterpret8/1 -> concatenate/8
  in9/1 -> reinterpret9/1
  reinterpret9/1 -> concatenate/9
  in10/1 -> reinterpret10/1
  reinterpret10/1 -> concatenate/10
  in11/1 -> reinterpret11/1
  reinterpret11/1 -> concatenate/11
  in12/1 -> reinterpret12/1
  reinterpret12/1 -> concatenate/12
  in13/1 -> reinterpret13/1
  reinterpret13/1 -> concatenate/13
  in14/1 -> reinterpret14/1
  reinterpret14/1 -> concatenate/14
  in15/1 -> reinterpret15/1
  reinterpret15/1 -> concatenate/15
  in16/1 -> reinterpret16/1
  reinterpret16/1 -> concatenate/16

== system snap_adc5g_spec/fft_wideband_real/fft_direct/butterfly0_0/bus_norm1/conv1 ==
  note: (ones_bit & 1) -> round-to-even
      | (ones_bit ^ 1) -> round-to-odd
      | (sign_bit & 1)-> round-to-zero
      | (sign_bit ^ 1) -> round-to-inf
      | (X ~| 1) -> round half down
      | (X | 1) -> round half up
  in : Inport
  Concat : xbsIndex_r4/Concat  num_inputs=2  dbl_ovrd=off  block_type=concat
      settings: block_version=10.1.3
  Constant : xbsIndex_r4/Constant  const=1  gui_display_data_type=Fixed-point  arith_type=Unsigned  n_bits=1  bin_pt=0  preci_type=Single  exp_width=8  frac_width=24  explicit_period=off  period=1  equ=P=C  opselect=C  inp2=PCIN>>17  opr=+  inp1=P  carry=CIN  dbl_ovrd=off  block_type=constant
  Reinterpret : xbsIndex_r4/Reinterpret  force_arith_type=on  arith_type=Unsigned  force_bin_pt=on  bin_pt=0  block_type=reinterpret
      settings: infoedit="Changes signal type without altering the binary representation.   You can changed the signal between signed and unsigned, and relocate the binary point.<P><P>Hardware notes: In hardware this block costs nothing.<P><P>Example:  Suppose the input is 6 bits wide, signed, with 2 fractional bits, and the output is forced to unsigned with 0 fractional bits.  Then an input of -2.0 (1110.00 in binary 2's complement) becomes an output of 56 (111000 in binary)."  block_version=10.1.3
  adder : xbsIndex_r4/AddSub  mode=Addition  use_carryin=off  use_carryout=off  en=off  latency=0  precision=User Defined  arith_type="Signed  (2's comp)"  n_bits=21  bin_pt=18  quantization=Truncate  overflow=Wrap  use_behavioral_HDL=off  hw_selection=Fabric  pipelined=on  use_rpm=on  dbl_ovrd=off  block_type=addsub
      settings: xl_area=[0, 0, 0, 0, 0, 0, 0]  block_version=10.1.3
  almost_half : xbsIndex_r4/Constant  const=0  gui_display_data_type=Fixed-point  arith_type=Unsigned  n_bits=19  bin_pt=0  preci_type=Single  exp_width=8  frac_width=24  explicit_period=off  period=1  equ=P=C  opselect=C  inp2=PCIN>>17  opr=+  inp1=P  carry=CIN  dbl_ovrd=off  block_type=constant
  bit : xbsIndex_r4/Slice  nbits=1  boolean_output=off  mode=Lower Bit Location + Width  bit1=0  base1=MSB of Input  bit0=0  base0=LSB of Input  dbl_ovrd=off  block_type=slice
      settings: infoedit="Extracts a given range of bits from each input sample and presents it at the output.  The output type is ordinarily unsigned with binary point at zero, but can be Boolean when the slice is one bit wide.<P><P>Hardware notes: In hardware this block costs nothing."  block_version=10.1.3
  force1 : xbsIndex_r4/Reinterpret  force_arith_type=on  arith_type="Signed  (2's comp)"  force_bin_pt=on  bin_pt=19  block_type=reinterpret
      settings: infoedit="Changes signal type without altering the binary representation.   You can changed the signal between signed and unsigned, and relocate the binary point.<P><P>Hardware notes: In hardware this block costs nothing.<P><P>Example:  Suppose the input is 6 bits wide, signed, with 2 fractional bits, and the output is forced to unsigned with 0 fractional bits.  Then an input of -2.0 (1110.00 in binary 2's complement) becomes an output of 56 (111000 in binary)."  block_version=10.1.3
  force2 : xbsIndex_r4/Reinterpret  force_arith_type=off  arith_type="Signed  (2's comp)"  force_bin_pt=on  bin_pt=19  block_type=reinterpret
      settings: infoedit="Changes signal type without altering the binary representation.   You can changed the signal between signed and unsigned, and relocate the binary point.<P><P>Hardware notes: In hardware this block costs nothing.<P><P>Example:  Suppose the input is 6 bits wide, signed, with 2 fractional bits, and the output is forced to unsigned with 0 fractional bits.  Then an input of -2.0 (1110.00 in binary 2's complement) becomes an output of 56 (111000 in binary)."  block_version=10.1.3
  tweak_op : xbsIndex_r4/Logical  logical_function=NOR  inputs=2  en=off  latency=0  precision=Full  arith_type=Unsigned  n_bits=8  bin_pt=2  align_bp=on  dbl_ovrd=off  block_type=logical
      settings: xl_area=[0, 0, 0, 0, 0, 0, 0]
  out : Outport
  wires:
  tweak_op/1 -> Concat/2
  Constant/1 -> tweak_op/2
  bit/1 -> tweak_op/1
  almost_half/1 -> force2/1
  in/1 -> Reinterpret/1, bit/1
  Concat/1 -> force1/1
  Reinterpret/1 -> Concat/1
  force1/1 -> adder/1
  force2/1 -> adder/2
  adder/1 -> out/1

== system snap_adc5g_spec/fft_wideband_real/fft_direct/butterfly0_0/bus_norm1/conv10 ==
  note: (ones_bit & 1) -> round-to-even
      | (ones_bit ^ 1) -> round-to-odd
      | (sign_bit & 1)-> round-to-zero
      | (sign_bit ^ 1) -> round-to-inf
      | (X ~| 1) -> round half down
      | (X | 1) -> round half up
  in : Inport
  Concat : xbsIndex_r4/Concat  num_inputs=2  dbl_ovrd=off  block_type=concat
      settings: block_version=10.1.3
  Constant : xbsIndex_r4/Constant  const=1  gui_display_data_type=Fixed-point  arith_type=Unsigned  n_bits=1  bin_pt=0  preci_type=Single  exp_width=8  frac_width=24  explicit_period=off  period=1  equ=P=C  opselect=C  inp2=PCIN>>17  opr=+  inp1=P  carry=CIN  dbl_ovrd=off  block_type=constant
  Reinterpret : xbsIndex_r4/Reinterpret  force_arith_type=on  arith_type=Unsigned  force_bin_pt=on  bin_pt=0  block_type=reinterpret
      settings: infoedit="Changes signal type without altering the binary representation.   You can changed the signal between signed and unsigned, and relocate the binary point.<P><P>Hardware notes: In hardware this block costs nothing.<P><P>Example:  Suppose the input is 6 bits wide, signed, with 2 fractional bits, and the output is forced to unsigned with 0 fractional bits.  Then an input of -2.0 (1110.00 in binary 2's complement) becomes an output of 56 (111000 in binary)."  block_version=10.1.3
  adder : xbsIndex_r4/AddSub  mode=Addition  use_carryin=off  use_carryout=off  en=off  latency=0  precision=User Defined  arith_type="Signed  (2's comp)"  n_bits=21  bin_pt=18  quantization=Truncate  overflow=Wrap  use_behavioral_HDL=off  hw_selection=Fabric  pipelined=on  use_rpm=on  dbl_ovrd=off  block_type=addsub
      settings: xl_area=[0, 0, 0, 0, 0, 0, 0]  block_version=10.1.3
  almost_half : xbsIndex_r4/Constant  const=0  gui_display_data_type=Fixed-point  arith_type=Unsigned  n_bits=19  bin_pt=0  preci_type=Single  exp_width=8  frac_width=24  explicit_period=off  period=1  equ=P=C  opselect=C  inp2=PCIN>>17  opr=+  inp1=P  carry=CIN  dbl_ovrd=off  block_type=constant
  bit : xbsIndex_r4/Slice  nbits=1  boolean_output=off  mode=Lower Bit Location + Width  bit1=0  base1=MSB of Input  bit0=0  base0=LSB of Input  dbl_ovrd=off  block_type=slice
      settings: infoedit="Extracts a given range of bits from each input sample and presents it at the output.  The output type is ordinarily unsigned with binary point at zero, but can be Boolean when the slice is one bit wide.<P><P>Hardware notes: In hardware this block costs nothing."  block_version=10.1.3
  force1 : xbsIndex_r4/Reinterpret  force_arith_type=on  arith_type="Signed  (2's comp)"  force_bin_pt=on  bin_pt=19  block_type=reinterpret
      settings: infoedit="Changes signal type without altering the binary representation.   You can changed the signal between signed and unsigned, and relocate the binary point.<P><P>Hardware notes: In hardware this block costs nothing.<P><P>Example:  Suppose the input is 6 bits wide, signed, with 2 fractional bits, and the output is forced to unsigned with 0 fractional bits.  Then an input of -2.0 (1110.00 in binary 2's complement) becomes an output of 56 (111000 in binary)."  block_version=10.1.3
  force2 : xbsIndex_r4/Reinterpret  force_arith_type=off  arith_type="Signed  (2's comp)"  force_bin_pt=on  bin_pt=19  block_type=reinterpret
      settings: infoedit="Changes signal type without altering the binary representation.   You can changed the signal between signed and unsigned, and relocate the binary point.<P><P>Hardware notes: In hardware this block costs nothing.<P><P>Example:  Suppose the input is 6 bits wide, signed, with 2 fractional bits, and the output is forced to unsigned with 0 fractional bits.  Then an input of -2.0 (1110.00 in binary 2's complement) becomes an output of 56 (111000 in binary)."  block_version=10.1.3
  tweak_op : xbsIndex_r4/Logical  logical_function=NOR  inputs=2  en=off  latency=0  precision=Full  arith_type=Unsigned  n_bits=8  bin_pt=2  align_bp=on  dbl_ovrd=off  block_type=logical
      settings: xl_area=[0, 0, 0, 0, 0, 0, 0]
  out : Outport
  wires:
  tweak_op/1 -> Concat/2
  Constant/1 -> tweak_op/2
  bit/1 -> tweak_op/1
  almost_half/1 -> force2/1
  in/1 -> Reinterpret/1, bit/1
  Concat/1 -> force1/1
  Reinterpret/1 -> Concat/1
  force1/1 -> adder/1
  force2/1 -> adder/2
  adder/1 -> out/1
